simulink model "PrmM_CustomerRequest"  (R2018b)
settings: Solver=FixedStepDiscrete  StartTime=0.0  StopTime=5  RelTol=1e-3  EnableMultiTasking=on
undefined symbols (not defined in the file): CS_PrmM_nHSpdBd_XDF32, CS_PrmM_nLwrSpdBd_XDF32
libraries: CalibrationLib x1
settings Model: DataDictionary=PrmM_Data.sldd  Creator=NWA2ST  LastModifiedBy=JYB2MC
settings DataIOCC: SaveFormat=StructureWithTime  SaveState=on  ReturnWorkspaceOutputs=on
settings OptimizationCC: BlockReduction=off  DefaultParameterBehavior=Inlined  UseDivisionForNetSlopeComputation=on  DefaultUnderspecifiedDataType=single  InlineInvariantSignals=on  BufferReuse=off  EnhancedBackFolding=on  GlobalBufferReuse=off  PassReuseOutputArgsAs=Individual arguments  PassReuseOutputArgsThreshold=6  RollThreshold=40  ActiveStateOutputEnumStorageType=uint8  ZeroExternalMemoryAtStartup=off  ZeroInternalMemoryAtStartup=off  EfficientFloat2IntCast=on  LifeSpan=inf  BufferReusableBoundary=off  OptimizeBlockOrder=speed  OptimizeDataStoreBuffers=off  LabelGuidedReuse=on
settings DebuggingCC: SignalInfNanChecking=error  SignalRangeChecking=error  ReadBeforeWriteMsg=EnableAllAsError  WriteAfterWriteMsg=EnableAllAsError  WriteAfterReadMsg=EnableAllAsError  AlgebraicLoopMsg=error  ArtificialAlgebraicLoopMsg=error  SaveWithDisabledLinksMsg=error  SaveWithParameterizedLinksMsg=error  BlockPriorityViolationMsg=error  SolverPrmCheckMsg=error  InheritedTsInSrcMsg=error  SingleTaskRateTransMsg=error  TasksWithSamePriorityMsg=error  SigSpecEnsureSampleTimeMsg=error  CheckMatrixSingularityMsg=error  IntegerOverflowMsg=error  ParameterUnderflowMsg=error  ParameterPrecisionLossMsg=error  ParameterTunabilityLossMsg=error  UnderSpecifiedDataTypeMsg=error  UnnecessaryDatatypeConvMsg=warning  VectorMatrixConversionMsg=error  SignalLabelMismatchMsg=error  UnconnectedInputMsg=error  UnconnectedOutputMsg=error  UnconnectedLineMsg=error  SFcnCompatibilityMsg=error  FrameProcessingCompatibilityMsg=warning  UniqueDataStoreMsg=error  BusObjectLabelMismatch=error  RootOutportRequireBusObject=error  AssertControl=DisableAll  AllowSymbolicDim=off  ModelReferenceIOMsg=error  ModelReferenceIOMismatchMessage=error  UnknownTsInhSupMsg=error  ModelReferenceDataLoggingMessage=error  StateNameClashWarn=warning  StrictBusMsg=ErrorOnBusTreatedAsVector  NonBusSignalsTreatedAsBus=error  SFInvalidInputDataAccessInChartInitDiag=error  SFTransitionOutsideNaturalParentDiag=error  SFUnreachableExecutionPathDiag=error  SFUndirectedBroadcastEventsDiag=error  SFTransitionActionBeforeConditionDiag=error  SFExecutionAtInitializationDiag=none  IntegerSaturationMsg=error
settings HardwareCC: ProdBitPerPointer=32  ProdBitPerSizeT=32  ProdBitPerPtrDiffT=32  ProdLargestAtomicInteger=Long  ProdWordSize=32  ProdHWDeviceType=Infineon->TriCore
settings ModelReferenceCC: EnableRefExpFcnMdlSchedulingChecks=off  EnableParallelModelReferenceBuilds=on  ModelReferenceNumInstancesAllowed=Single  PropagateSignalLabelsOutOfModel=off
settings SFSimCC: SimCustomHeaderCode="#include \"Rte_Type.h\""  SimUserIncludeDirs="\"include\""  SFSimEcho=off  SimParseCustomCode=off  SimGenImportedTypeDefs=on  CompileTimeRecursionLimit=0  EnableRuntimeRecursion=off  MATLABDynamicMemAlloc=off
settings RTWCC: SystemTargetFile=autosar.tlc  GenCodeOnly=on  TemplateMakefile=ert_default_tmf  PostCodeGenCommand=SEGPostCodeGenCallback(modelName, buildInfo)  Description=AUTOSAR  IncludeHyperlinkInReport=on
settings RTWCC: CustomInclude=|
  | ..\..\..\..\03_SrvLyr\SysSrv\StdT\cfg\Cfg_Output\manual
  | ..\..\..\..\02_Rte\Ecu_cfg\cfg\Cfg_Output\generated
  | ..\..\..\..\03_SrvLyr\SysSrv\OS\cfg\Cfg_Output\generated
settings CodeAppCC: ForceParamTrailComments=on  CommentStyle=Single-line  IgnoreCustomStorageClasses=off  IgnoreTestpoints=on  MangleLength=4  SharedChecksumLength=4  CustomSymbolStrGlobalVar=$U$R$N$M  CustomSymbolStrType=$R_$N$M  CustomSymbolStrFcn=$U$R_$N$F$M  CustomSymbolStrFcnArg=$U$N$M_$I[l]  CustomSymbolStrBlkIO=$N$M  CustomUserTokenString=CS  ReqsInCode=on
settings STFCustomTargetCC: TargetLangStandard=C99 (ISO)  UtilityFuncGeneration=Shared location  MultiwordLength=256  ParMdlRefBuildCompliant=on  CompOptLevelCompliant=on  IncludeMdlTerminateFcn=off  CombineOutputUpdateFcns=on  CombineSignalStateStructs=on  SuppressErrorStatus=on  ERTCustomFileBanners=on  SupportAbsoluteTime=off  SupportNonFinite=off  SupportComplex=off  SupportContinuousTime=off  SupportNonInlinedSFcns=off  ParenthesesLevel=Maximum  CastingMode=Standards  MATLABClassNameForMDSCustomization=Simulink.SoftwareTarget.ERTCustomization  AutosarCompliant=on  UseToolchainInfoCompliant=on  GenerateSharedConstants=off  LookupTableObjectStructAxisOrder=2,1,3,4,...  LUTObjectStructOrderEvenSpacing=Size,Table,Breakpoints  SystemTargetFile=autosar.tlc
settings ERTTargetCC: TargetLangStandard=C99 (ISO)  UtilityFuncGeneration=Shared location  ConcurrentExecutionCompliant=off  IncludeMdlTerminateFcn=off  CombineSignalStateStructs=on  SuppressErrorStatus=on  SupportAbsoluteTime=off  SupportNonFinite=off  SupportComplex=off  RemoveResetFunc=off  ParenthesesLevel=Maximum  CastingMode=Standards  ModelStepFunctionPrototypeControlCompliant=off  CPPClassGenCompliant=off  AutosarCompliant=on  GenerateSharedConstants=off  LookupTableObjectStructAxisOrder=2,1,3,4,...  LUTObjectStructOrderEvenSpacing=Size,Table,Breakpoints  GenerateASAP2=on  InlinedParameterPlacement=NonHierarchical  ERTSrcFileBannerTemplate=ert_code_template_SEG_EEB_R2018b.cgt  ERTHdrFileBannerTemplate=ert_code_template_SEG_EEB_R2018b.cgt  ERTDataSrcFileTemplate=ert_code_template_SEG_EEB_R2018b.cgt  ERTDataHdrFileTemplate=ert_code_template_SEG_EEB_R2018b.cgt  ERTCustomFileTemplate=example_file_process_SEG_EEB_R2018b.tlc  PreserveExpressionOrder=on  PreserveIfCondition=on  ConvertIfToSwitch=off  SuppressUnreachableDefaultCases=off  EnableSignedLeftShifts=off  EnableSignedRightShifts=off  BooleanTrueId=TRUE  BooleanFalseId=FALSE  TypeLimitIdReplacementHeaderFile=Platform_Types.h  MemSecPackage=arMemmap  MemSecDataConstants=CONST_UNSPECIFIED  MemSecDataIO=VAR_UNSPECIFIED  MemSecDataInternal=VAR_UNSPECIFIED  MemSecDataParameters=CONST_UNSPECIFIED  MemSecFuncInitTerm=CODE  MemSecFuncExecute=CODE  MemSecFuncSharedUtil=CODE

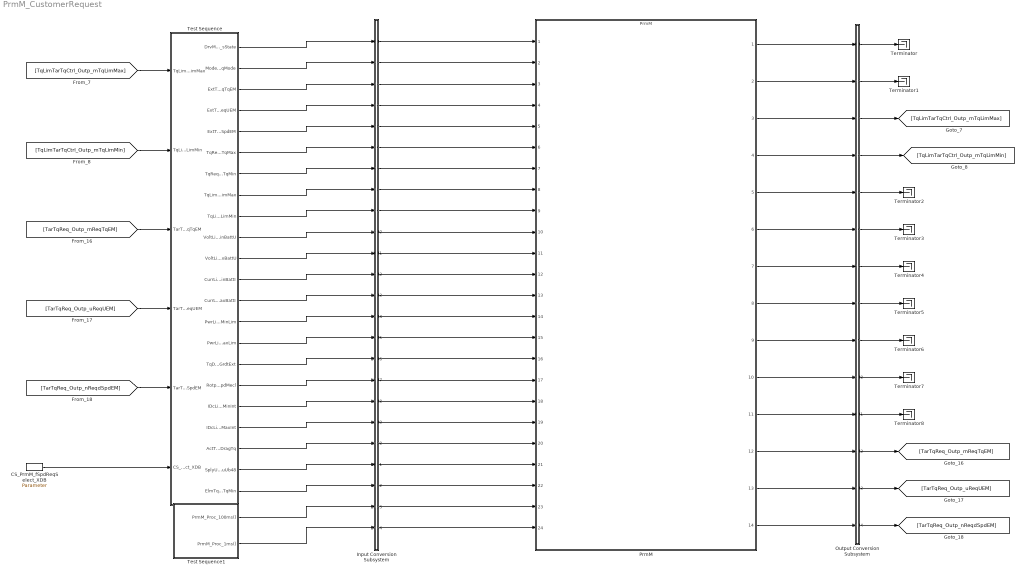
== system PrmM_CustomerRequest ==
  CS_PrmM_fSpdReqSelect_XDB : CalibrationLib/Parameter  calParamName=CS_PrmM_fSpdReqSelect_XDB
      settings: AttributesFormatString=%<calParamName>  SourceProductName=SEG Calibration Lib
  Input Conversion Subsystem : Subsystem  Tag=__SLT_ICS__  Description=|
      | Signal spec.
      | and routing
      settings: AttributesFormatString=%<Description>
  Output Conversion Subsystem : Subsystem  Tag=__SLT_OCS__  Description=|
      | Signal spec.
      | and routing
      settings: AttributesFormatString=%<Description>
  PrmM : ModelReference  ModelNameDialog=PrmM  SimulationMode=Normal  CodeInterface=Top model  ModelReferenceVersion=1.16
  Terminator{,1..8} (9 alike) : Terminator
  Test Sequence : Test Sequence  TreatAsAtomicUnit=on
  Test Sequence1 : Test Sequence  TreatAsAtomicUnit=on
  wires:
  [TqLimTarTqCtrl_Outp_mTqLimMin] -> Test Sequence/2(TqLimTarTqCtrl_Outp_mTqLimMin)
  [TqLimTarTqCtrl_Outp_mTqLimMax] -> Test Sequence/1(TqLimTarTqCtrl_Outp_mTqLimMax)
  [TarTqReq_Outp_nReqdSpdEM] -> Test Sequence/5(TarTqReq_Outp_nReqdSpdEM)
  [TarTqReq_Outp_uReqUEM] -> Test Sequence/4(TarTqReq_Outp_uReqUEM)
  [TarTqReq_Outp_mReqTqEM] -> Test Sequence/3(TarTqReq_Outp_mReqTqEM)
  CS_PrmM_fSpdReqSelect_XDB/1 -> Test Sequence/6(CS_PrmM_fSpdReqSelect_XDB)
  PrmM/1 -> Output Conversion Subsystem/1(Inport_1)
  PrmM/2 -> Output Conversion Subsystem/2(Inport_2)
  PrmM/3 -> Output Conversion Subsystem/3(Inport_3)
  PrmM/4 -> Output Conversion Subsystem/4(Inport_4)
  PrmM/5 -> Output Conversion Subsystem/5(Inport_5)
  PrmM/6 -> Output Conversion Subsystem/6(Inport_6)
  PrmM/7 -> Output Conversion Subsystem/7(Inport_7)
  PrmM/8 -> Output Conversion Subsystem/8(Inport_8)
  PrmM/9 -> Output Conversion Subsystem/9(Inport_9)
  PrmM/10 -> Output Conversion Subsystem/10(Inport_10)
  PrmM/11 -> Output Conversion Subsystem/11(Inport_11)
  PrmM/12 -> Output Conversion Subsystem/12(Inport_12)
  PrmM/13 -> Output Conversion Subsystem/13(Inport_13)
  PrmM/14 -> Output Conversion Subsystem/14(Inport_14)
  Input Conversion Subsystem/1(Outport_1) -> PrmM/1
  Input Conversion Subsystem/2(Outport_2) -> PrmM/2
  Input Conversion Subsystem/3(Outport_3) -> PrmM/3
  Input Conversion Subsystem/4(Outport_4) -> PrmM/4
  Input Conversion Subsystem/5(Outport_5) -> PrmM/5
  Input Conversion Subsystem/6(Outport_6) -> PrmM/6
  Input Conversion Subsystem/7(Outport_7) -> PrmM/7
  Input Conversion Subsystem/8(Outport_8) -> PrmM/8
  Input Conversion Subsystem/9(Outport_9) -> PrmM/9
  Input Conversion Subsystem/10(Outport_10) -> PrmM/10
  Input Conversion Subsystem/11(Outport_11) -> PrmM/11
  Input Conversion Subsystem/12(Outport_12) -> PrmM/12
  Input Conversion Subsystem/13(Outport_13) -> PrmM/13
  Input Conversion Subsystem/14(Outport_14) -> PrmM/14
  Input Conversion Subsystem/15(Outport_15) -> PrmM/15
  Input Conversion Subsystem/16(Outport_16) -> PrmM/16
  Input Conversion Subsystem/17(Outport_17) -> PrmM/17
  Input Conversion Subsystem/18(Outport_18) -> PrmM/18
  Input Conversion Subsystem/19(Outport_19) -> PrmM/19
  Input Conversion Subsystem/20(Outport_20) -> PrmM/20
  Input Conversion Subsystem/21(Outport_21) -> PrmM/21
  Input Conversion Subsystem/22(Outport_22) -> PrmM/22
  Input Conversion Subsystem/23(Outport_23) -> PrmM/23
  Input Conversion Subsystem/24(Outport_24) -> PrmM/24
  Output Conversion Subsystem/1(Outport_1) -> Terminator/1
  Output Conversion Subsystem/2(Outport_2) -> Terminator1/1
  Output Conversion Subsystem/14(Outport_14) -> [TarTqReq_Outp_nReqdSpdEM]
  Output Conversion Subsystem/13(Outport_13) -> [TarTqReq_Outp_uReqUEM]
  Output Conversion Subsystem/12(Outport_12) -> [TarTqReq_Outp_mReqTqEM]
  Output Conversion Subsystem/11(Outport_11) -> Terminator8/1
  Output Conversion Subsystem/10(Outport_10) -> Terminator7/1
  Output Conversion Subsystem/9(Outport_9) -> Terminator6/1
  Output Conversion Subsystem/8(Outport_8) -> Terminator5/1
  Output Conversion Subsystem/7(Outport_7) -> Terminator4/1
  Output Conversion Subsystem/6(Outport_6) -> Terminator3/1
  Output Conversion Subsystem/5(Outport_5) -> Terminator2/1
  Output Conversion Subsystem/4(Outport_4) -> [TqLimTarTqCtrl_Outp_mTqLimMin]
  Output Conversion Subsystem/3(Outport_3) -> [TqLimTarTqCtrl_Outp_mTqLimMax]
  Test Sequence1/1(PrmM_Proc_100ms()) -> Input Conversion Subsystem/23(Inport_23)
  Test Sequence1/2(PrmM_Proc_1ms()) -> Input Conversion Subsystem/24(Inport_24)
  Test Sequence/1(DrvM_Inp_sState) -> Input Conversion Subsystem/1(Inport_1)
  Test Sequence/2(ModeReqInt_Inp_sIntReqMode) -> Input Conversion Subsystem/2(Inport_2)
  Test Sequence/3(ExtTarTqReq_Inp_mReqTqEM) -> Input Conversion Subsystem/3(Inport_3)
  Test Sequence/4(ExtTarTqReq_Inp_uReqUEM) -> Input Conversion Subsystem/4(Inport_4)
  Test Sequence/5(ExtTarTqReq_Inp_nReqdSpdEM) -> Input Conversion Subsystem/5(Inport_5)
  Test Sequence/6(TqReqLim_Inp_mTqMax) -> Input Conversion Subsystem/6(Inport_6)
  Test Sequence/7(TqReqLim_Inp_mTqMin) -> Input Conversion Subsystem/7(Inport_7)
  Test Sequence/8(TqLimExt_Inp_mTqLimMax) -> Input Conversion Subsystem/8(Inport_8)
  Test Sequence/9(TqLimExt_Inp_mTqLimMin) -> Input Conversion Subsystem/9(Inport_9)
  Test Sequence/10(VoltLimExt_Inp_uReqdMinBattU) -> Input Conversion Subsystem/10(Inport_10)
  Test Sequence/11(VoltLimExt_Inp_uReqdMaxBattU) -> Input Conversion Subsystem/11(Inport_11)
  Test Sequence/12(CurrLimExt_Inp_iReqdMinBattI) -> Input Conversion Subsystem/12(Inport_12)
  Test Sequence/13(CurrLimExt_Inp_iReqdMaxBattI) -> Input Conversion Subsystem/13(Inport_13)
  Test Sequence/14(PwrLimExt_Inp_pPwrMinLim) -> Input Conversion Subsystem/14(Inport_14)
  Test Sequence/15(PwrLimExt_Inp_pPwrMaxLim) -> Input Conversion Subsystem/15(Inport_15)
  Test Sequence/16(TqDesGrdtExt_Inp_TqDesGrdtExt) -> Input Conversion Subsystem/16(Inport_16)
  Test Sequence/17(Rotp_Inp_nSpdMecl) -> Input Conversion Subsystem/17(Inport_17)
  Test Sequence/18(IDcLim_Inp_IDcLimMinInt) -> Input Conversion Subsystem/18(Inport_18)
  Test Sequence/19(IDcLim_Inp_IDcLimMaxInt) -> Input Conversion Subsystem/19(Inport_19)
  Test Sequence/20(ActTq_Inp_mDragTq) -> Input Conversion Subsystem/20(Inport_20)
  Test Sequence/21(SplyU48_uUb48) -> Input Conversion Subsystem/21(Inport_21)
  Test Sequence/22(ElmTqLim_mTqMin) -> Input Conversion Subsystem/22(Inport_22)

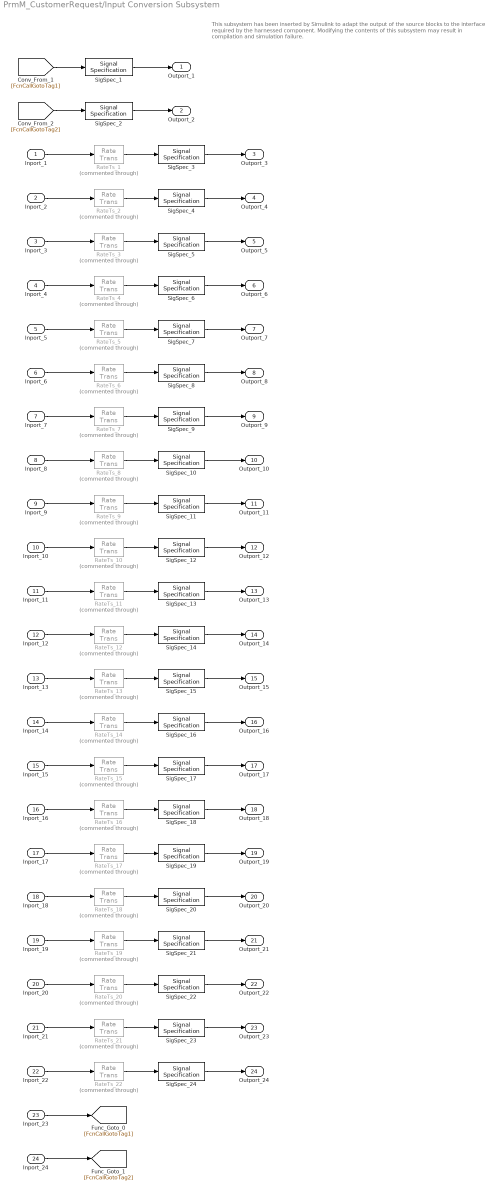
== system PrmM_CustomerRequest/Input Conversion Subsystem ==
  note: This subsystem has been inserted by Simulink to adapt the output of the source blocks to the interface required by the harnessed component.
      |  Modifying the contents of this subsystem may result in compilation and simulation failure.
  Inport_1 : Inport
  Inport_2 : Inport  Port=2
  Inport_3 : Inport  Port=3
  Inport_4 : Inport  Port=4
  Inport_5 : Inport  Port=5
  Inport_6 : Inport  Port=6
  Inport_7 : Inport  Port=7
  Inport_8 : Inport  Port=8
  Inport_9 : Inport  Port=9
  Inport_10 : Inport  Port=10
  Inport_11 : Inport  Port=11
  Inport_12 : Inport  Port=12
  Inport_13 : Inport  Port=13
  Inport_14 : Inport  Port=14
  Inport_15 : Inport  Port=15
  Inport_16 : Inport  Port=16
  Inport_17 : Inport  Port=17
  Inport_18 : Inport  Port=18
  Inport_19 : Inport  Port=19
  Inport_20 : Inport  Port=20
  Inport_21 : Inport  Port=21
  Inport_22 : Inport  Port=22
  Inport_23 : Inport  Port=23
  Inport_24 : Inport  Port=24
  RateTs_{1..22} (22 alike) : RateTransition  Commented=through
  SigSpec_1 : SignalSpecification
  SigSpec_10 : SignalSpecification  OutDataTypeStr=AD_tMTQLIMMAXEXT  Unit=N*m  Dimensions=[1]
  SigSpec_11 : SignalSpecification  OutDataTypeStr=AD_tMTQLIMMINEXT  Unit=N*m  Dimensions=[1]
  SigSpec_12 : SignalSpecification  OutDataTypeStr=AD_tUVOLTMINLIMEXT  Dimensions=[1]
  SigSpec_13 : SignalSpecification  OutDataTypeStr=AD_tUVOLTMAXLIMEXT  Dimensions=[1]
  SigSpec_14 : SignalSpecification  OutDataTypeStr=AD_tICURRMINLIMEXT  Dimensions=[1]
  SigSpec_15 : SignalSpecification  OutDataTypeStr=AD_tICURRMAXLIMEXT  Dimensions=[1]
  SigSpec_16 : SignalSpecification  OutDataTypeStr=AD_tPPWRMINLIMEXT  Dimensions=[1]
  SigSpec_17 : SignalSpecification  OutDataTypeStr=AD_tPPWRMAXLIMEXT  Dimensions=[1]
  SigSpec_18 : SignalSpecification  OutDataTypeStr=AD_tYTQGRDTLIMEXT  Dimensions=[1]
  SigSpec_19 : SignalSpecification  OutDataTypeStr=AD_RotP_tNSPDMECL  Dimensions=[1]
  SigSpec_2 : SignalSpecification
  SigSpec_20 : SignalSpecification  OutDataTypeStr=AD_tIDCLIMMININT  Dimensions=[1]
  SigSpec_21 : SignalSpecification  OutDataTypeStr=AD_tIDCLIMMAXINT  Dimensions=[1]
  SigSpec_22 : SignalSpecification  OutDataTypeStr=AD_ActTq_tMDRAGTQ  Dimensions=[1]
  SigSpec_23 : SignalSpecification  OutDataTypeStr=AD_SplyU_tUUB48  Dimensions=[1]
  SigSpec_24 : SignalSpecification  OutDataTypeStr=AD_ElmTqLim_tMTQMIN  Dimensions=[1]
  SigSpec_3 : SignalSpecification  OutDataTypeStr=Enum: AD_DrvM_tSTATEIDX_E  Dimensions=[1]
  SigSpec_4 : SignalSpecification  OutDataTypeStr=Enum: AD_DrvM_tSTATEIDX_E  Dimensions=[1]
  SigSpec_5 : SignalSpecification  OutDataTypeStr=AD_tMREQTQEMEXT  Dimensions=[1]
  SigSpec_6 : SignalSpecification  OutDataTypeStr=AD_tUREQVOLTEMEXT  Dimensions=[1]
  SigSpec_7 : SignalSpecification  OutDataTypeStr=AD_tNREQDSPDEMEXT  Dimensions=[1]
  SigSpec_8 : SignalSpecification  OutDataTypeStr=AD_TqReqLim_tMTQMAX  Dimensions=[1]
  SigSpec_9 : SignalSpecification  OutDataTypeStr=AD_TqReqLim_tMTQMIN  Dimensions=[1]
  Outport_1 : Outport
  Outport_2 : Outport  Port=2
  Outport_3 : Outport  Port=3
  Outport_4 : Outport  Port=4
  Outport_5 : Outport  Port=5
  Outport_6 : Outport  Port=6
  Outport_7 : Outport  Port=7
  Outport_8 : Outport  Port=8
  Outport_9 : Outport  Port=9
  Outport_10 : Outport  Port=10
  Outport_11 : Outport  Port=11
  Outport_12 : Outport  Port=12
  Outport_13 : Outport  Port=13
  Outport_14 : Outport  Port=14
  Outport_15 : Outport  Port=15
  Outport_16 : Outport  Port=16
  Outport_17 : Outport  Port=17
  Outport_18 : Outport  Port=18
  Outport_19 : Outport  Port=19
  Outport_20 : Outport  Port=20
  Outport_21 : Outport  Port=21
  Outport_22 : Outport  Port=22
  Outport_23 : Outport  Port=23
  Outport_24 : Outport  Port=24
  wires:
  SigSpec_1/1 -> Outport_1/1
  [FcnCallGotoTag1] -> SigSpec_1/1
  SigSpec_2/1 -> Outport_2/1
  [FcnCallGotoTag2] -> SigSpec_2/1
  SigSpec_3/1 -> Outport_3/1
  RateTs_1/1 -> SigSpec_3/1
  Inport_1/1 -> RateTs_1/1
  SigSpec_4/1 -> Outport_4/1
  RateTs_2/1 -> SigSpec_4/1
  Inport_2/1 -> RateTs_2/1
  SigSpec_5/1 -> Outport_5/1
  RateTs_3/1 -> SigSpec_5/1
  Inport_3/1 -> RateTs_3/1
  SigSpec_6/1 -> Outport_6/1
  RateTs_4/1 -> SigSpec_6/1
  Inport_4/1 -> RateTs_4/1
  SigSpec_7/1 -> Outport_7/1
  RateTs_5/1 -> SigSpec_7/1
  Inport_5/1 -> RateTs_5/1
  SigSpec_8/1 -> Outport_8/1
  RateTs_6/1 -> SigSpec_8/1
  Inport_6/1 -> RateTs_6/1
  SigSpec_9/1 -> Outport_9/1
  RateTs_7/1 -> SigSpec_9/1
  Inport_7/1 -> RateTs_7/1
  SigSpec_10/1 -> Outport_10/1
  RateTs_8/1 -> SigSpec_10/1
  Inport_8/1 -> RateTs_8/1
  SigSpec_11/1 -> Outport_11/1
  RateTs_9/1 -> SigSpec_11/1
  Inport_9/1 -> RateTs_9/1
  SigSpec_12/1 -> Outport_12/1
  RateTs_10/1 -> SigSpec_12/1
  Inport_10/1 -> RateTs_10/1
  SigSpec_13/1 -> Outport_13/1
  RateTs_11/1 -> SigSpec_13/1
  Inport_11/1 -> RateTs_11/1
  SigSpec_14/1 -> Outport_14/1
  RateTs_12/1 -> SigSpec_14/1
  Inport_12/1 -> RateTs_12/1
  SigSpec_15/1 -> Outport_15/1
  RateTs_13/1 -> SigSpec_15/1
  Inport_13/1 -> RateTs_13/1
  SigSpec_16/1 -> Outport_16/1
  RateTs_14/1 -> SigSpec_16/1
  Inport_14/1 -> RateTs_14/1
  SigSpec_17/1 -> Outport_17/1
  RateTs_15/1 -> SigSpec_17/1
  Inport_15/1 -> RateTs_15/1
  SigSpec_18/1 -> Outport_18/1
  RateTs_16/1 -> SigSpec_18/1
  Inport_16/1 -> RateTs_16/1
  SigSpec_19/1 -> Outport_19/1
  RateTs_17/1 -> SigSpec_19/1
  Inport_17/1 -> RateTs_17/1
  SigSpec_20/1 -> Outport_20/1
  RateTs_18/1 -> SigSpec_20/1
  Inport_18/1 -> RateTs_18/1
  SigSpec_21/1 -> Outport_21/1
  RateTs_19/1 -> SigSpec_21/1
  Inport_19/1 -> RateTs_19/1
  SigSpec_22/1 -> Outport_22/1
  RateTs_20/1 -> SigSpec_22/1
  Inport_20/1 -> RateTs_20/1
  SigSpec_23/1 -> Outport_23/1
  RateTs_21/1 -> SigSpec_23/1
  Inport_21/1 -> RateTs_21/1
  SigSpec_24/1 -> Outport_24/1
  RateTs_22/1 -> SigSpec_24/1
  Inport_22/1 -> RateTs_22/1
  Inport_23/1 -> [FcnCallGotoTag1]
  Inport_24/1 -> [FcnCallGotoTag2]

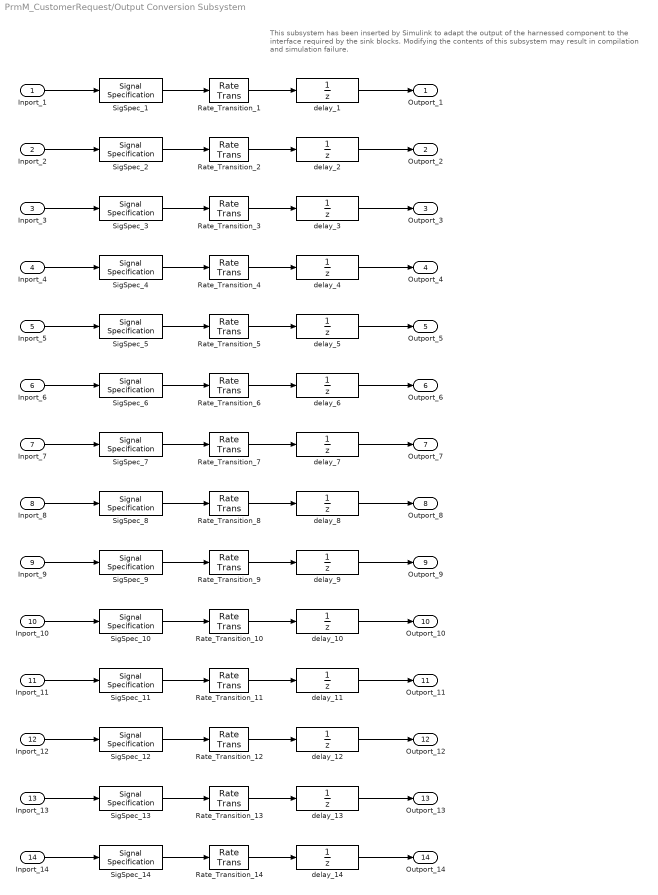
== system PrmM_CustomerRequest/Output Conversion Subsystem ==
  note: This subsystem has been inserted by Simulink to adapt the output of the harnessed component to the interface required by the sink blocks.
      |  Modifying the contents of this subsystem may result in compilation and simulation failure.
  Inport_1 : Inport
  Inport_2 : Inport  Port=2
  Inport_3 : Inport  Port=3
  Inport_4 : Inport  Port=4
  Inport_5 : Inport  Port=5
  Inport_6 : Inport  Port=6
  Inport_7 : Inport  Port=7
  Inport_8 : Inport  Port=8
  Inport_9 : Inport  Port=9
  Inport_10 : Inport  Port=10
  Inport_11 : Inport  Port=11
  Inport_12 : Inport  Port=12
  Inport_13 : Inport  Port=13
  Inport_14 : Inport  Port=14
  Rate_Transition_{1..14} (14 alike) : RateTransition  OutPortSampleTimeOpt=Inherit
  SigSpec_1 : SignalSpecification  OutDataTypeStr=AD_PrmM_tUDCMINALLWD  Dimensions=[1]
  SigSpec_10 : SignalSpecification  OutDataTypeStr=AD_ComWrp_tPPWRMINLIM  Dimensions=[1]
  SigSpec_11 : SignalSpecification  OutDataTypeStr=AD_ComWrp_tPPWRMAXLIM  Dimensions=[1]
  SigSpec_12 : SignalSpecification  OutDataTypeStr=AD_ComWrp_tMREQTQEM  Unit=N*m  Dimensions=[1]
  SigSpec_13 : SignalSpecification  OutDataTypeStr=AD_ComWrp_tUREQVOLTEM  Unit=V  Dimensions=[1]
  SigSpec_14 : SignalSpecification  OutDataTypeStr=AD_ComWrp_tNREQDSPDEM  Unit=rpm  Dimensions=[1]
  SigSpec_2 : SignalSpecification  OutDataTypeStr=AD_PrmM_tUDCMAXALLWD  Dimensions=[1]
  SigSpec_3 : SignalSpecification  OutDataTypeStr=AD_ComWrp_tMTQLIMMAX  Unit=N*m  Dimensions=[1]
  SigSpec_4 : SignalSpecification  OutDataTypeStr=AD_ComWrp_tMTQLIMMIN  Unit=N*m  Dimensions=[1]
  SigSpec_5 : SignalSpecification  OutDataTypeStr=AD_PrmM_tMMAXTQGRDINT  Unit=N*m/s  Dimensions=[1]
  SigSpec_6 : SignalSpecification  OutDataTypeStr=AD_ComWrp_tIREQDMINBATTI  Unit=A  Dimensions=[1]
  SigSpec_7 : SignalSpecification  OutDataTypeStr=AD_ComWrp_tIREQDMAXBATTI  Unit=A  Dimensions=[1]
  SigSpec_8 : SignalSpecification  OutDataTypeStr=AD_ComWrp_tUREQDMINBATTU  Unit=V  Dimensions=[1]
  SigSpec_9 : SignalSpecification  OutDataTypeStr=AD_ComWrp_tUREQDMAXBATTU  Unit=V  Dimensions=[1]
  delay_{1..14} (14 alike) : UnitDelay  SampleTime=-1
  Outport_1 : Outport
  Outport_2 : Outport  Port=2
  Outport_3 : Outport  Port=3
  Outport_4 : Outport  Port=4
  Outport_5 : Outport  Port=5
  Outport_6 : Outport  Port=6
  Outport_7 : Outport  Port=7
  Outport_8 : Outport  Port=8
  Outport_9 : Outport  Port=9
  Outport_10 : Outport  Port=10
  Outport_11 : Outport  Port=11
  Outport_12 : Outport  Port=12
  Outport_13 : Outport  Port=13
  Outport_14 : Outport  Port=14
  wires:
  Inport_1/1 -> SigSpec_1/1
  SigSpec_1/1 -> Rate_Transition_1/1
  Rate_Transition_1/1 -> delay_1/1
  delay_1/1 -> Outport_1/1
  Inport_2/1 -> SigSpec_2/1
  SigSpec_2/1 -> Rate_Transition_2/1
  Rate_Transition_2/1 -> delay_2/1
  delay_2/1 -> Outport_2/1
  Inport_3/1 -> SigSpec_3/1
  SigSpec_3/1 -> Rate_Transition_3/1
  Rate_Transition_3/1 -> delay_3/1
  delay_3/1 -> Outport_3/1
  Inport_4/1 -> SigSpec_4/1
  SigSpec_4/1 -> Rate_Transition_4/1
  Rate_Transition_4/1 -> delay_4/1
  delay_4/1 -> Outport_4/1
  Inport_5/1 -> SigSpec_5/1
  SigSpec_5/1 -> Rate_Transition_5/1
  Rate_Transition_5/1 -> delay_5/1
  delay_5/1 -> Outport_5/1
  Inport_6/1 -> SigSpec_6/1
  SigSpec_6/1 -> Rate_Transition_6/1
  Rate_Transition_6/1 -> delay_6/1
  delay_6/1 -> Outport_6/1
  Inport_7/1 -> SigSpec_7/1
  SigSpec_7/1 -> Rate_Transition_7/1
  Rate_Transition_7/1 -> delay_7/1
  delay_7/1 -> Outport_7/1
  Inport_8/1 -> SigSpec_8/1
  SigSpec_8/1 -> Rate_Transition_8/1
  Rate_Transition_8/1 -> delay_8/1
  delay_8/1 -> Outport_8/1
  Inport_9/1 -> SigSpec_9/1
  SigSpec_9/1 -> Rate_Transition_9/1
  Rate_Transition_9/1 -> delay_9/1
  delay_9/1 -> Outport_9/1
  Inport_10/1 -> SigSpec_10/1
  SigSpec_10/1 -> Rate_Transition_10/1
  Rate_Transition_10/1 -> delay_10/1
  delay_10/1 -> Outport_10/1
  Inport_11/1 -> SigSpec_11/1
  SigSpec_11/1 -> Rate_Transition_11/1
  Rate_Transition_11/1 -> delay_11/1
  delay_11/1 -> Outport_11/1
  Inport_12/1 -> SigSpec_12/1
  SigSpec_12/1 -> Rate_Transition_12/1
  Rate_Transition_12/1 -> delay_12/1
  delay_12/1 -> Outport_12/1
  Inport_13/1 -> SigSpec_13/1
  SigSpec_13/1 -> Rate_Transition_13/1
  Rate_Transition_13/1 -> delay_13/1
  delay_13/1 -> Outport_13/1
  Inport_14/1 -> SigSpec_14/1
  SigSpec_14/1 -> Rate_Transition_14/1
  Rate_Transition_14/1 -> delay_14/1
  delay_14/1 -> Outport_14/1

== stateflow chart PrmM_CustomerRequest/Test Sequence1 ==
  settings: updateMethod=DISCRETE  sampleTime=0.001  stateMachineType=SIMPLIFIED_MACHINE
  state Run
    send(PrmM_Proc_1ms);
    if t == 0 || every(100, tick)
    send(PrmM_Proc_100ms);
    end
  (default) -> Run
  events: PrmM_Proc_100ms output FUNCTION_CALL_EVENT; PrmM_Proc_1ms output FUNCTION_CALL_EVENT

== stateflow chart PrmM_CustomerRequest/Test Sequence ==
  settings: updateMethod=DISCRETE  sampleTime=0.001  stateMachineType=SIMPLIFIED_MACHINE
  state Run
    %% Initialize data outputs.
    DrvM_Inp_sState = AD_DrvM_tSTATEIDX_E.CS_DrvM_STATE_Idle;
    ModeReqInt_Inp_sIntReqMode = AD_DrvM_tSTATEIDX_E.CS_DrvM_STATE_Idle;
    VoltLimExt_Inp_uReqdMinBattU = single(0);
    TqReqLim_Inp_mTqMax = single(65);
    TqReqLim_Inp_mTqMin = single(-65);
    VoltLimExt_Inp_uReqdMaxBattU = single(0);
    PwrLimExt_Inp_pPwrMinLim = single(0);
    PwrLimExt_Inp_pPwrMaxLim = single(0);
    TqDesGrdtExt_Inp_TqDesGrdtExt = single(0);
    Rotp_Inp_nSpdMecl = single(0);
    CurrLimExt_Inp_iReqdMinBattI = single(0);
    ExtTarTqReq_Inp_mReqTqEM = single(0);
    TqLimExt_Inp_mTqLimMin = single(-65);
    CurrLimExt_Inp_iReqdMaxBattI = single(0);
    TqLimExt_Inp_mTqLimMax = single(65);
    ExtTarTqReq_Inp_nReqdSpdEM = single(0);
    ExtTarTqReq_Inp_uReqUEM = single(0);
    ActTq_Inp_mDragTq = single(0.3);
    IDcLim_Inp_IDcLimMinInt=single(-290);
    IDcLim_Inp_IDcLimMaxInt=single(360);
    ElmTqLim_mTqMin=single(-60);
    SplyU48_uUb48=single(48);
  state ChooseDesiredRequest
    state TorqueMode
      DrvM_Inp_sState = AD_DrvM_tSTATEIDX_E.CS_DrvM_STATE_Tq;
      ModeReqInt_Inp_sIntReqMode = AD_DrvM_tSTATEIDX_E.CS_DrvM_STATE_Tq;
      ExtTarTqReq_Inp_mReqTqEM=single(10)
      state wait
      state verfiy
        verify(abs(TarTqReq_Outp_mReqTqEM-ExtTarTqReq_Inp_mReqTqEM)<Tolerance)
      (default) -> ChooseDesiredRequest.TorqueMode.wait
      ChooseDesiredRequest.TorqueMode.wait -> ChooseDesiredRequest.TorqueMode.verfiy : [after(0.1,sec)
          | ]
    state SpeedMode
      DrvM_Inp_sState = AD_DrvM_tSTATEIDX_E.CS_DrvM_STATE_Spd;
      ExtTarTqReq_Inp_nReqdSpdEM=single(2000)
      state ExternalRequestIsChosen
        state wait
        state verfiy
          verify(abs(TarTqReq_Outp_nReqdSpdEM-ExtTarTqReq_Inp_nReqdSpdEM)<Tolerance)
        (default) -> ChooseDesiredRequest.SpeedMode.ExternalRequestIsChosen.wait
        ChooseDesiredRequest.SpeedMode.ExternalRequestIsChosen.wait -> ChooseDesiredRequest.SpeedMode.ExternalRequestIsChosen.verfiy : [(CS_PrmM_fSpdReqSelect_XDB==true)&&after(0.1,sec)
            | ]
      state InternalRequestIsChosen
        state wait
        state verfiy
          verify(abs(TarTqReq_Outp_nReqdSpdEM-single(0))<Tolerance)
        (default) -> ChooseDesiredRequest.SpeedMode.InternalRequestIsChosen.wait
        ChooseDesiredRequest.SpeedMode.InternalRequestIsChosen.wait -> ChooseDesiredRequest.SpeedMode.InternalRequestIsChosen.verfiy : [after(0.1,sec)
            | ]
      (default) -> ExternalRequestIsChosen
      ExternalRequestIsChosen -> InternalRequestIsChosen : [CS_PrmM_fSpdReqSelect_XDB==false
          | ]
    state VoltageMode
      DrvM_Inp_sState = AD_DrvM_tSTATEIDX_E.CS_DrvM_STATE_Volt;
      ExtTarTqReq_Inp_uReqUEM=single(48)
      Rotp_Inp_nSpdMecl = single(CS_PrmM_nHSpdBd_XDF32+1);
      state wait
      state verfiy
        verify(abs(TarTqReq_Outp_uReqUEM-ExtTarTqReq_Inp_uReqUEM)<Tolerance)
        verify(abs(TqLimTarTqCtrl_Outp_mTqLimMin-TqReqLim_Inp_mTqMin)<Tolerance)
        verify(abs(TqLimTarTqCtrl_Outp_mTqLimMax+ActTq_Inp_mDragTq)<Tolerance)
      (default) -> ChooseDesiredRequest.VoltageMode.wait
      ChooseDesiredRequest.VoltageMode.wait -> ChooseDesiredRequest.VoltageMode.verfiy : [after(0.1,sec)
          | ]
    state CommuincationlossMode
      DrvM_Inp_sState = AD_DrvM_tSTATEIDX_E.CS_DrvM_STATE_ComLoss
      ExtTarTqReq_Inp_uReqUEM=single(48)
      Rotp_Inp_nSpdMecl=single(CS_PrmM_nLwrSpdBd_XDF32-1)
      state wait
      state verfiy
        verify(abs(TarTqReq_Outp_uReqUEM-single(45))<Tolerance)
        verify(abs(TqLimTarTqCtrl_Outp_mTqLimMin+ActTq_Inp_mDragTq)<Tolerance)
        verify(abs(TqLimTarTqCtrl_Outp_mTqLimMax+ActTq_Inp_mDragTq)<Tolerance)
        verify(abs(TarTqReq_Outp_mReqTqEM+ActTq_Inp_mDragTq)<Tolerance)
      (default) -> ChooseDesiredRequest.CommuincationlossMode.wait
      ChooseDesiredRequest.CommuincationlossMode.wait -> ChooseDesiredRequest.CommuincationlossMode.verfiy : [after(0.1,sec)
          | ]
    state CommuincationlossMode1
      DrvM_Inp_sState = AD_DrvM_tSTATEIDX_E.CS_DrvM_STATE_ComLoss
      ExtTarTqReq_Inp_uReqUEM=single(48)
      Rotp_Inp_nSpdMecl=single(CS_PrmM_nLwrSpdBd_XDF32+1)
      intpl_TqMin=(TqReqLim_Inp_mTqMin +ActTq_Inp_mDragTq)*(Rotp_Inp_nSpdMecl-CS_PrmM_nLwrSpdBd_XDF32)/(CS_PrmM_nHSpdBd_XDF32-CS_PrmM_nLwrSpdBd_XDF32)-ActTq_Inp_mDragTq
      state wait
      state verfiy
        verify(abs(TarTqReq_Outp_uReqUEM-single(45))<Tolerance)
        verify(abs(TqLimTarTqCtrl_Outp_mTqLimMin-intpl_TqMin)<Tolerance)
        verify(abs(TqLimTarTqCtrl_Outp_mTqLimMax+ActTq_Inp_mDragTq)<Tolerance)
      (default) -> ChooseDesiredRequest.CommuincationlossMode1.wait
      ChooseDesiredRequest.CommuincationlossMode1.wait -> ChooseDesiredRequest.CommuincationlossMode1.verfiy : [after(0.1,sec)
          | ]
    state BatteryDisconnecedMode
      DrvM_Inp_sState = AD_DrvM_tSTATEIDX_E.CS_DrvM_STATE_BattDiscnctd;
      if after(0.002,sec)
      ExtTarTqReq_Inp_uReqUEM=single(52)
      elseif after(0.001,sec)
      ExtTarTqReq_Inp_uReqUEM=single(45)
      else
      ExtTarTqReq_Inp_uReqUEM=single(23)
      end
      state wait
      state verfiy
        verify(abs(TqLimTarTqCtrl_Outp_mTqLimMax+ActTq_Inp_mDragTq)<Tolerance)
        verify(abs(TarTqReq_Outp_uReqUEM-single(51))<Tolerance)
      (default) -> ChooseDesiredRequest.BatteryDisconnecedMode.wait
      ChooseDesiredRequest.BatteryDisconnecedMode.wait -> ChooseDesiredRequest.BatteryDisconnecedMode.verfiy : [after(0.1,sec)
          | ]
    (default) -> TorqueMode
    TorqueMode -> SpeedMode : [after(0.5,sec)
        | ]
    SpeedMode -> VoltageMode : [after(1,sec)
        | ]
    VoltageMode -> CommuincationlossMode : [after(0.5,sec)
        | ]
    CommuincationlossMode -> CommuincationlossMode1 : [after(0.5,sec)
        | ]
    CommuincationlossMode1 -> BatteryDisconnecedMode : [after(0.5,sec)
        | ]
  (default) -> Run
  Run -> ChooseDesiredRequest
  data: TqLimTarTqCtrl_Outp_mTqLimMax input AD_ComWrp_tMTQLIMMAX size=[1]; TqLimTarTqCtrl_Outp_mTqLimMin input AD_ComWrp_tMTQLIMMIN size=[1]; TarTqReq_Outp_mReqTqEM input AD_ComWrp_tMREQTQEM size=[1]; TarTqReq_Outp_uReqUEM input AD_ComWrp_tUREQVOLTEM size=[1]; TarTqReq_Outp_nReqdSpdEM input AD_ComWrp_tNREQDSPDEM size=[1]; DrvM_Inp_sState output Enum: AD_DrvM_tSTATEIDX_E size=[1]; ModeReqInt_Inp_sIntReqMode output Enum: AD_DrvM_tSTATEIDX_E size=[1]; ExtTarTqReq_Inp_mReqTqEM output AD_ComWrp_tMREQTQEM size=[1]; ExtTarTqReq_Inp_uReqUEM output AD_ComWrp_tUREQVOLTEM size=[1]; ExtTarTqReq_Inp_nReqdSpdEM output AD_ComWrp_tNREQDSPDEM size=[1]; TqReqLim_Inp_mTqMax output AD_TqReqLim_tMTQMAX size=[1]; TqReqLim_Inp_mTqMin output AD_TqReqLim_tMTQMIN size=[1]; TqLimExt_Inp_mTqLimMax output AD_ComWrp_tMTQLIMMAX size=[1]; TqLimExt_Inp_mTqLimMin output AD_ComWrp_tMTQLIMMIN size=[1]; VoltLimExt_Inp_uReqdMinBattU output AD_ComWrp_tUREQDMINBATTU size=[1]; VoltLimExt_Inp_uReqdMaxBattU output AD_ComWrp_tUREQDMAXBATTU size=[1]; CurrLimExt_Inp_iReqdMinBattI output AD_ComWrp_tIREQDMINBATTI size=[1]; CurrLimExt_Inp_iReqdMaxBattI output AD_ComWrp_tIREQDMAXBATTI size=[1]; PwrLimExt_Inp_pPwrMinLim output AD_ComWrp_tPPWRMINLIM size=[1]; PwrLimExt_Inp_pPwrMaxLim output AD_ComWrp_tPPWRMAXLIM size=[1]; TqDesGrdtExt_Inp_TqDesGrdtExt output AD_tYTQGRDTLIMEXT size=[1]; Rotp_Inp_nSpdMecl output AD_RotP_tNSPDMECL size=[1]; IDcLim_Inp_IDcLimMinInt output; IDcLim_Inp_IDcLimMaxInt output; ActTq_Inp_mDragTq output AD_ActTq_tMDRAGTQ size=[1]; SplyU48_uUb48 output; Tolerance constant single =0.01; CS_PrmM_fSpdReqSelect_XDB input; ElmTqLim_mTqMin output; CS_PrmM_nLwrSpdBd_XDF32 parameter; CS_PrmM_nHSpdBd_XDF32 parameter; intpl_TqMin local
